simulink model "M1_Starter_PI_Only"  (R2026a)
settings: Solver=ode15s  StopTime=2  MaxStep=0.001
settings Model: Creator=siddh  LastModifiedBy=sjawahar

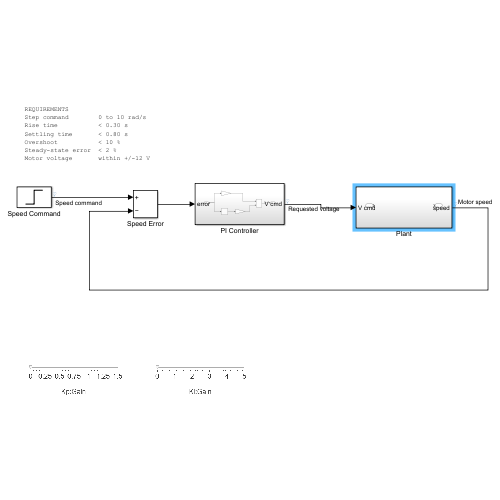
[thumbnail: Simulink's stored preview of the top-level diagram]
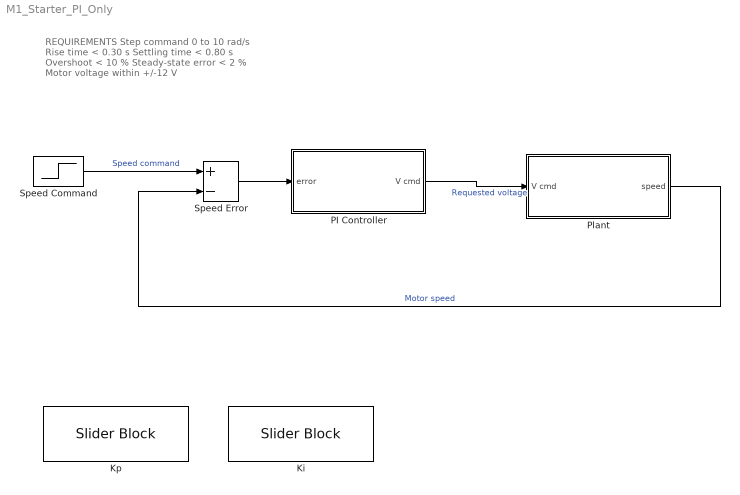
== system M1_Starter_PI_Only ==
  note: REQUIREMENTS
      | Step command        0 to 10 rad/s
      | Rise time           < 0.30 s
      | Settling time       < 0.80 s
      | Overshoot           < 10 %
      | Steady-state error  < 2 %
      | Motor voltage       within +/-12 V
  Ki : SliderBlock  LabelPosition=Bottom  ScaleMax=5
  Kp : SliderBlock  LabelPosition=Bottom  ScaleMax=1.5
  PI Controller : Subsystem
  Plant : Subsystem
  Speed Command : Step  Time=0.1  FinalValue=10  SampleTime=0
  Speed Error : Sum  Inputs=+-
  wires:
  Speed Command/1 -> Speed Error/1  "Speed command"
  Speed Error/1 -> PI Controller/1(error)
  PI Controller/1(V cmd) -> Plant/1(V cmd)  "Requested voltage"
  Plant/1(speed) -> Speed Error/2  "Motor speed"

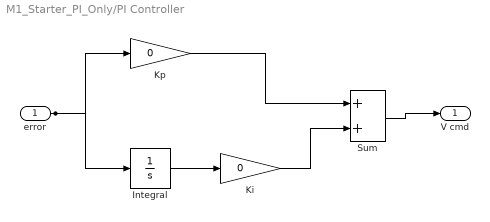
== system M1_Starter_PI_Only/PI Controller ==
  error : Inport
  Integral : Integrator
  Ki : Gain  Gain=0
  Kp : Gain  Gain=0
  Sum : Sum
  V cmd : Outport
  wires:
  error/1 -> Kp/1, Integral/1
  Integral/1 -> Ki/1
  Kp/1 -> Sum/1
  Ki/1 -> Sum/2
  Sum/1 -> V cmd/1

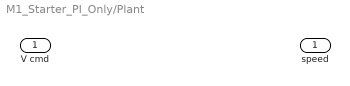
== system M1_Starter_PI_Only/Plant ==
  V cmd : Inport
  speed : Outport
